simulink model "Reformable_AI_2025"  (R2025b)
settings: Solver=ode23t  StartTime=0.0  StopTime=150  FixedStep=0.01  RelTol=1e-3
InitFcn:
  | load('PV_Params_Stage1.mat'); load('PV_Params_Stage2.mat');
values from neighbouring files (symbols this model uses):
  Iph_ref = P.Iph_ref*(1 - K.k_Iph*D)    [PaperFigures.m]
  n = lower(name)    [Stage10C_inventory.m]    (also in Stage10F2_make_manifest.m = size(rows,1); Stage10F_make_manifest.m = size(rows,1); Stage10F_run_one.m = 1; Stage10_assemble_dataset.m = height(T))
  OCV_tbl = [11.6 11.8 11.9 12.1 12.2 12.3 12.4 12.5 12.6 12.7 12.8]    [Battery_Param_Definition.m]
  Q = 7    [Battery_Param_Definition.m]
  q = 1.602176634e-19    [PaperFigures.m]    (also in Stage10C_inventory.m = L(strcmp({L.folder}, fl{k})); Stage10F2_make_manifest.m = M(M.regime == "A" & abs(M.bD - L) < 1e-12, :); Stage10F_make_manifest.m = M(M.regime == "A" & abs(M.bD - L) < 1e-12, :); Stage10G2_final_test.m = zeros(1, numel(seeds)))
  R0 = 0.03    [Battery_Param_Definition.m]    (also in PaperFigures.m = B.R0*(1 + KB.k_R0*D))
  R1 = 0.015    [Battery_Param_Definition.m]    (also in PaperFigures.m = B.R1*(1 + KB.k_R1*D))
  Rs = P.Rs*(1 + K.k_Rs*D)    [PaperFigures.m]
  Rsh = P.Rsh*(1 - K.k_Rsh*D)    [PaperFigures.m]
  SOC_bp = [0 10 20 30 40 50 60 70 80 90 100]    [Battery_Param_Definition.m]
  SOC_init = 100    [Battery_Param_Definition.m]
undefined symbols (not defined in the file or in its folder): Battery_Twin_C1, Battery_Twin_Capacity, Battery_Twin_OCV_tbl, Battery_Twin_R0, Battery_Twin_R1, Battery_Twin_SOC_bp, Battery_Twin_SOC_init, Battery_Twin_Vp_init, bias_G, bias_I_batt, bias_I_pv, bias_T_batt, bias_Tc, bias_V_batt, bias_V_pv, dG, dI_batt, dI_pv, drift_G, drift_I_batt, drift_I_pv, drift_T_batt, drift_Tc, drift_V_batt, drift_V_pv, dT_batt, dTc, dV_batt, dV_pv, Eg, ExcessiveNoise_Sigma, ExcessiveNoise_Sigma_batt, ExtraDrift_Rate, ExtraDrift_Rate_batt, FaultBias_Value, FaultBias_Value_batt, FaultSat_Max, FaultSat_Max_batt, FaultSat_Min, FaultSat_Min_batt, G_max, G_min, Gref, I0_ref, I_batt_max, I_batt_min, I_pv_max, I_pv_min, IntermittentDropoutProb, IntermittentDropoutProb_batt, Isc_ref, k_B, k_Iph, k_Q, k_R0, k_R1, k_Rs, k_Rsh, Ki, noise_G ... (+44)
libraries: fl_lib x7, nesl_utility x6
(part 3 of 3)

== matlab function Reformable_AI_2025/PV_Rolling_Features/MATLAB Function ==
  settings: updateMethod=DISCRETE
  data: t input; PV_Residual_Current_Mean output; PV_Residual_Current input; PV_Residual_Power input; PV_Residual_Current_Std output; PV_Residual_Current_MaxAbs output; PV_Residual_Power_Mean output; PV_Residual_Power_Std output; PV_Residual_Power_MaxAbs output; PV_Feature_Window_Valid output; Stage9_Window_Short parameter; Stage9_Window_Medium parameter; Stage9_Max_Buffer_Samples parameter; PV_Residual_Current_Trend output; PV_Residual_Power_Trend output; PV_Trend_Window_Valid output; Stage9_Window_Long parameter
function [PV_Residual_Current_Mean, PV_Residual_Current_Std, PV_Residual_Current_MaxAbs, ...
          PV_Residual_Power_Mean, PV_Residual_Power_Std, PV_Residual_Power_MaxAbs, ...
          PV_Feature_Window_Valid, ...
          PV_Residual_Current_Trend, PV_Residual_Power_Trend, PV_Trend_Window_Valid] = ...
    fcn(t, PV_Residual_Current, PV_Residual_Power, ...
        Stage9_Window_Short, Stage9_Window_Medium, Stage9_Max_Buffer_Samples, Stage9_Window_Long)

% TwinAdapt-PHM Stage 9 (Step 2+3): PV_Feature_Engineering -- Group C + D
% Group C (rolling mean/std/max) unchanged from the verified version.
% Group D (trend/slope) added here, reusing the SAME buffer -- no reason
% to duplicate a second buffer just to compute a slope over the data
% we're already holding.
%
% Trend = least-squares slope of residual vs time over Stage9_Window_Long,
% using CENTERED time (t - mean(t) within the window) per Stage 9 Section
% 17's explicit numerical-stability requirement -- a naive slope formula
% using raw (large) simulation-time values would be ill-conditioned.
%
% NOTE ON SYMBOLS PANE: t, PV_Residual_Current, PV_Residual_Power must be
% Scope = Input. Stage9_Window_Short, Stage9_Window_Medium,
% Stage9_Window_Long, Stage9_Max_Buffer_Samples must be Scope = Parameter.
% (Stage9_Window_Long is a NEW addition to this block's Symbols pane --
% add it as Parameter, same as the other three.)
%
% Give this block itself a discrete Sample Time of Stage9_Feature_SampleTime
% in its Block Parameters dialog (NOT the Symbols pane) -- required
% because ode23t is an implicit variable-step solver that evaluates
% trial/rejected time points internally; without a fixed sample time this
% block's persistent buffer gets corrupted by those non-real trial calls.

persistent buf_t buf_I buf_P

if isempty(buf_t)
    buf_t = nan(1, Stage9_Max_Buffer_Samples);
    buf_I = nan(1, Stage9_Max_Buffer_Samples);
    buf_P = nan(1, Stage9_Max_Buffer_Samples);
end

% --- Shift buffer left by one, append newest sample at the end.
% Fixed size in, fixed size out -- every single call. ---
buf_t = [buf_t(2:end), t];
buf_I = [buf_I(2:end), PV_Residual_Current];
buf_P = [buf_P(2:end), PV_Residual_Power];

% ===================== Group C: rolling mean/std/max =====================
maskMedium = (t - buf_t) <= Stage9_Window_Medium;
maskShort  = (t - buf_t) <= Stage9_Window_Short;

IWinMedium = buf_I; IWinMedium(~maskMedium) = NaN;
PWinMedium = buf_P; PWinMedium(~maskMedium) = NaN;
IWinShort  = buf_I; IWinShort(~maskShort)   = NaN;
PWinShort  = buf_P; PWinShort(~maskShort)   = NaN;

PV_Residual_Current_Mean = mean(IWinMedium, 'omitnan');
PV_Residual_Current_Std  = std(IWinMedium, 0, 'omitnan');
PV_Residual_Power_Mean   = mean(PWinMedium, 'omitnan');
PV_Residual_Power_Std    = std(PWinMedium, 0, 'omitnan');

PV_Residual_Current_MaxAbs = max(abs(IWinShort), [], 'omitnan');
PV_Residual_Power_MaxAbs   = max(abs(PWinShort), [], 'omitnan');

oldestRealTime = min(buf_t);
if isnan(oldestRealTime)
    PV_Feature_Window_Valid = false;
else
    PV_Feature_Window_Valid = (t - oldestRealTime) >= Stage9_Window_Medium;
end

% ===================== Group D: trend (centered-time slope) =====================
maskLong = (t - buf_t) <= Stage9_Window_Long;

tWinLong = buf_t; tWinLong(~maskLong) = NaN;
IWinLong = buf_I; IWinLong(~maskLong) = NaN;
PWinLong = buf_P; PWinLong(~maskLong) = NaN;

tCentered = tWinLong - mean(tWinLong, 'omitnan');   % NaN stays NaN, correctly excluded downstream
ICentered = IWinLong - mean(IWinLong, 'omitnan');
PCentered = PWinLong - mean(PWinLong, 'omitnan');

denom = sum(tCentered.^2, 'omitnan');

if denom > eps   % guard against divide-by-zero when the window holds too few distinct points
    PV_Residual_Current_Trend = sum(tCentered .* ICentered, 'omitnan') / denom;
    PV_Residual_Power_Trend   = sum(tCentered .* PCentered, 'omitnan') / denom;
else
    PV_Residual_Current_Trend = 0;
    PV_Residual_Power_Trend   = 0;
end

if isnan(oldestRealTime)
    PV_Trend_Window_Valid = false;
else
    PV_Trend_Window_Valid = (t - oldestRealTime) >= Stage9_Window_Long;
end

end

== matlab function Reformable_AI_2025/PV_Twin_Valid_Operating_Point/MATLAB Function ==
  data: PV_Measured_Voltage input; PV_Twin_Valid_Operating_Point output; PV_Measured_Irradiance input; PV_Twin_Current input; PV_Twin_Power input; Stage9_PV_Voltage_Min parameter; Stage9_PV_Voltage_Max parameter; Stage9_Min_Irradiance parameter
function PV_Twin_Valid_Operating_Point = ...
    fcn(PV_Measured_Voltage, PV_Measured_Irradiance, PV_Twin_Current, PV_Twin_Power, ...
        Stage9_PV_Voltage_Min, Stage9_PV_Voltage_Max, Stage9_Min_Irradiance)

% TwinAdapt-PHM Stage 9 (Step 4): PV_Twin_Valid_Operating_Point
% This flag does NOT fix PV_Digital_Twin's Newton-Raphson domain
% limitation (Stage 8 Section 46: do not modify Stage 8 for this). It
% identifies when the Twin's inputs/outputs fall outside the domain the
% Twin was validated for, so later PHM stages can discount or ignore a
% residual computed under those conditions rather than mistaking solver
% breakdown for genuine physical degradation.
%
% Checks, per Stage 9 Section 19:
%   - measured voltage within [Stage9_PV_Voltage_Min, Stage9_PV_Voltage_Max]
%     (the Max threshold is 0.95*Voc_ref -- the documented Stage 8 Test 6
%     boundary where the solve starts diverging)
%   - measured irradiance above the meaningful-generation threshold
%     (same Stage9_Min_Irradiance used in Group A -- reused, not
%     redefined, since it's the same physical justification)
%   - Twin outputs are finite (catches any other solver breakdown not
%     already caught by the voltage check)
%   - Twin current is non-negative (a diode model producing negative
%     current in this regime is itself a sign of a bad solve)
%
% This is metadata/context, not a fault label (Stage 9 Section 20) --
% it says "trust this residual less right now," not "something is wrong
% with the physical asset."
%
% NOTE ON SYMBOLS PANE: PV_Measured_Voltage, PV_Measured_Irradiance,
% PV_Twin_Current, PV_Twin_Power must be Scope = Input. The three
% threshold parameters must be Scope = Parameter.

voltageInRange = (PV_Measured_Voltage >= Stage9_PV_Voltage_Min) && ...
                 (PV_Measured_Voltage <= Stage9_PV_Voltage_Max);

irradianceMeaningful = PV_Measured_Irradiance >= Stage9_Min_Irradiance;

outputsFinite = isfinite(PV_Twin_Current) && isfinite(PV_Twin_Power);

currentPhysical = PV_Twin_Current >= 0;

PV_Twin_Valid_Operating_Point = voltageInRange && irradianceMeaningful && ...
                                 outputsFinite && currentPhysical;

end

== matlab function Reformable_AI_2025/Battery_Residual_Voltage/MATLAB Function ==
  data: Battery_Residual_Voltage input; Battery_AbsResidual_Voltage output; Battery_Normalized_Voltage_Residual output; Battery_V_nominal parameter
function [Battery_AbsResidual_Voltage, Battery_Normalized_Voltage_Residual] = ...
    fcn(Battery_Residual_Voltage, Battery_V_nominal)

% TwinAdapt-PHM Stage 9 (Step 5): Battery_Feature_Engineering -- Group A+B
% Mirrors PV_Feature_Engineering Step 1, scaled down to match what
% actually exists upstream: only ONE battery residual (voltage) exists,
% since Battery_Digital_Twin never produces a current/power prediction
% (Stage 8 design decision -- current is the Twin's INPUT, not something
% it forecasts). No extra features manufactured just for PV/Battery
% symmetry.
%
% Normalization denominator (Battery_V_nominal) is a FIXED reference
% (max of the battery's own OCV table), never a live signal -- same
% safety reasoning as PV's Isc_ref/Pmax_ref.
%
% Deployment-observable: yes. Uses only the residual plus a fixed
% reference constant, no hidden ground truth.
%
% NOTE ON SYMBOLS PANE: Battery_Residual_Voltage must be Scope = Input.
% Battery_V_nominal must be Scope = Parameter.

Battery_AbsResidual_Voltage = abs(Battery_Residual_Voltage);
Battery_Normalized_Voltage_Residual = Battery_Residual_Voltage / Battery_V_nominal;

end

== matlab function Reformable_AI_2025/Battery_Feature_Engineering_2/MATLAB Function ==
  data: t input; Battery_Residual_Voltage_Mean output; Battery_Residual_Voltage input; Battery_Residual_Voltage_Std output; Battery_Residual_Voltage_MaxAbs output; Battery_Feature_Window_Valid output; Stage9_Window_Short parameter; Stage9_Window_Medium parameter; Stage9_Max_Buffer_Samples parameter; Battery_Residual_Voltage_Trend output; Battery_Trend_Window_Valid output; Stage9_Window_Long parameter
function [Battery_Residual_Voltage_Mean, Battery_Residual_Voltage_Std, ...
          Battery_Residual_Voltage_MaxAbs, Battery_Feature_Window_Valid, ...
          Battery_Residual_Voltage_Trend, Battery_Trend_Window_Valid] = ...
    fcn(t, Battery_Residual_Voltage, ...
        Stage9_Window_Short, Stage9_Window_Medium, Stage9_Max_Buffer_Samples, Stage9_Window_Long)

% TwinAdapt-PHM Stage 9: Battery_Feature_Engineering -- Group C + D
% Group C (verified) unchanged. Group D (trend) added, reusing the same
% buffer -- identical mechanism to PV_Rolling_Features' Group D: centered-
% time least-squares slope over Stage9_Window_Long, numerically stable
% regardless of the simulation's absolute time values.
%
% Sample Time for this block must remain set to Stage9_Feature_SampleTime
% in its Block Parameters dialog (carries over automatically since this
% is the same block, just with more code -- no need to re-set it).
%
% NOTE ON SYMBOLS PANE: Stage9_Window_Long is a NEW addition -- add it to
% this block's Symbols pane as Scope = Parameter (not Input), same as the
% other three window/buffer parameters.

persistent buf_t buf_V

if isempty(buf_t)
    buf_t = nan(1, Stage9_Max_Buffer_Samples);
    buf_V = nan(1, Stage9_Max_Buffer_Samples);
end

buf_t = [buf_t(2:end), t];
buf_V = [buf_V(2:end), Battery_Residual_Voltage];

% ===================== Group C: rolling mean/std/max =====================
maskMedium = (t - buf_t) <= Stage9_Window_Medium;
maskShort  = (t - buf_t) <= Stage9_Window_Short;

VWinMedium = buf_V; VWinMedium(~maskMedium) = NaN;
VWinShort  = buf_V; VWinShort(~maskShort)   = NaN;

Battery_Residual_Voltage_Mean   = mean(VWinMedium, 'omitnan');
Battery_Residual_Voltage_Std    = std(VWinMedium, 0, 'omitnan');
Battery_Residual_Voltage_MaxAbs = max(abs(VWinShort), [], 'omitnan');

oldestRealTime = min(buf_t);
if isnan(oldestRealTime)
    Battery_Feature_Window_Valid = false;
else
    Battery_Feature_Window_Valid = (t - oldestRealTime) >= Stage9_Window_Medium;
end

% ===================== Group D: trend (centered-time slope) =====================
maskLong = (t - buf_t) <= Stage9_Window_Long;

tWinLong = buf_t; tWinLong(~maskLong) = NaN;
VWinLong = buf_V; VWinLong(~maskLong) = NaN;

tCentered = tWinLong - mean(tWinLong, 'omitnan');
VCentered = VWinLong - mean(VWinLong, 'omitnan');

denom = sum(tCentered.^2, 'omitnan');

if denom > eps
    Battery_Residual_Voltage_Trend = sum(tCentered .* VCentered, 'omitnan') / denom;
else
    Battery_Residual_Voltage_Trend = 0;
end

if isnan(oldestRealTime)
    Battery_Trend_Window_Valid = false;
else
    Battery_Trend_Window_Valid = (t - oldestRealTime) >= Stage9_Window_Long;
end

end

== matlab function Reformable_AI_2025/PV_Degradation_Model/MATLAB Function ==
  data: t input; Rs_aged output; Rs_ref input; Rsh_ref input; Iph_ref_ref input; T_life input; k_Rs input; k_Rsh input; k_Iph input; Rsh_aged output; Iph_ref_aged output; D_index output; H_PV output; Health_State output

function [Rs_aged, Rsh_aged, Iph_ref_aged, D_index, H_PV, Health_State] = PV_Aging_Model(t, Rs_ref, Rsh_ref, Iph_ref_ref, T_life, k_Rs, k_Rsh, k_Iph)
%#codegen

D_index = min(1, t / T_life);

Rs_aged      = Rs_ref * (1 + k_Rs * D_index);
Rsh_aged     = Rsh_ref * (1 - k_Rsh * D_index);
Iph_ref_aged = Iph_ref_ref * (1 - k_Iph * D_index);

H_PV = 1 - D_index;

% Discrete health state classification (1=Healthy ... 5=Critical)
if D_index < 0.2
    Health_State = 1;   % Healthy
elseif D_index < 0.4
    Health_State = 2;   % Early Degradation
elseif D_index < 0.6
    Health_State = 3;   % Moderate Degradation
elseif D_index < 0.8
    Health_State = 4;   % Severe Degradation
else
    Health_State = 5;   % Critical
end

end

== matlab function Reformable_AI_2025/PV_model/MATLAB Function ==
  data: G input; I output; Tc_C input; V input; Rs input; P output; Rsh input; Iph_ref input; I0_ref input; n input; Ns input; Ki input; Eg input; Gref input; Tref input
function [I, P] = PV_SingleDiode_Solver(G, Tc_C, V, Rs, Rsh, Iph_ref, I0_ref, n, Ns, Ki, Eg, Gref, Tref)
%#codegen

k = 1.380649e-23;
q = 1.602176634e-19;

Tc = Tc_C + 273.15;
Vt = Ns*k*Tc/q;

Iph = (Iph_ref + Ki*(Tc - Tref)) * (G/Gref);
I0  = I0_ref * (Tc/Tref)^3 * exp((q*Eg/(n*k)) * (1/Tref - 1/Tc));

I = Iph;
for iter = 1:50
    expTerm = exp(min((V + I*Rs)/(n*Vt), 700));
    f  = Iph - I0*(expTerm - 1) - (V + I*Rs)/Rsh - I;
    df = -I0*(Rs/(n*Vt))*expTerm - Rs/Rsh - 1;
    dI = f/df;
    I  = I - dI;
    if abs(dI) < 1e-8
        break;
    end
end

I = max(I, 0);
P = V * I;
end

== matlab function Reformable_AI_2025/Battery_Degradation_Model/MATLAB Function ==
  data: t input; R0_aged output; R0_ref input; R1_ref input; Capacity_ref input; T_life input; k_R0 input; k_R1 input; k_Q input; R1_aged output; Capacity_aged output; OCV_deltaV output; D_batt output; H_batt output; Battery_Health_State output
function [R0_aged, R1_aged, Capacity_aged, OCV_deltaV, D_batt, H_batt, Battery_Health_State] = ...
    Battery_Aging_Model(t, R0_ref, R1_ref, Capacity_ref, T_life, k_R0, k_R1, k_Q)
%#codegen

D_batt = min(1, t / T_life);

R0_aged       = R0_ref * (1 + k_R0 * D_batt);
R1_aged       = R1_ref * (1 + k_R1 * D_batt);
Capacity_aged = Capacity_ref * (1 - k_Q * D_batt);

% Small, gradual OCV shift — capped so it never causes a sudden collapse
OCV_deltaV = 0.05 * D_batt;   % up to 50 mV shift at end-of-life; tune if needed

H_batt = 1 - D_batt;

% Discrete health state classification (1=Healthy ... 5=Critical)
if D_batt < 0.2
    Battery_Health_State = 1;
elseif D_batt < 0.4
    Battery_Health_State = 2;
elseif D_batt < 0.6
    Battery_Health_State = 3;
elseif D_batt < 0.8
    Battery_Health_State = 4;
else
    Battery_Health_State = 5;
end

end
